simulink model "sf_clutch_enabled_subsystems"  (R2025b)
settings: Solver=ode23  StartTime=0.0  StopTime=10  RelTol=1e-6  AbsTol=1e-7
model workspace (MATLAB code in the model file + MAT data in the model file):
  Fn = [0  0; 1  0.8; 2  1.6; 3  1.6; 4  1.6; 5  1.6; 6  0.8; 7  0; 8  0; 9  0; 10  0]
  Ie = 1
  Iv = 5
  R = 1
  Tin = [1  2; 2  2; 3  2; 4  2; 5  2; 6  0; 7  0; 8  0; 9  0; 10  0]
  be = 2
  bv = 1
  f1 = [1; 6; 11; 16; 21; 26; 31; 36; 41; 46; 51]
  muk = 1
  mus = 1.5
  other statements: load sldemo_clutchparam;
settings Model: ExtModeTrigMode=oneshot  ExtModeArmWhenConnect=off  ExtModeAutoUpdateStatusClock=off  Creator=The MathWorks, Inc.  LastModifiedBy=The MathWorks, Inc.
settings SolverCC: AutoScaleAbsTol=off  AlgebraicLoopSolver=TrustRegion  InsertRTBMode=Auto
settings DataIOCC: ExternalInput=[]  InitialState=[]  SaveFormat=Array  SaveOutput=off  SaveTime=off  ReturnWorkspaceOutputs=off  StateSaveName=x  TimeSaveName=t  OutputSaveName=y  SignalLoggingName=sldemo_clutch_output
settings OptimizationCC: BlockReduction=off  BooleanDataType=off  ReuseModelBlockBuffer=off  ExpressionDepthLimit=2147483647.0  InitFltsAndDblsToZero=on  EfficientMapNaN2IntZero=off  LifeSpan=inf  BufferReusableBoundary=off
settings DebuggingCC: SaveWithParameterizedLinksMsg=none  UnderspecifiedInitializationDetection=Classic  MergeDetectMultiDrivingBlocksExec=none  SignalResolutionControl=TryResolveAllWithWarning  MultiTaskDSMMsg=warning  MultiTaskCondExecSysMsg=none  SigSpecEnsureSampleTimeMsg=none  IntegerOverflowMsg=none  FcnCallInpInsideContextMsg=warning  UnconnectedInputMsg=warning  UnconnectedOutputMsg=warning  UnconnectedLineMsg=warning  BusObjectLabelMismatch=none  StateNameClashWarn=warning  SFUnexpectedBacktrackingDiag=warning  SFNoUnconditionalDefaultTransitionDiag=warning  SFExecutionAtInitializationDiag=none  IntegerSaturationMsg=none  ArithmeticOperatorsInVariantConditions=warning
settings HardwareCC: ProdBitPerPointer=32.0  ProdBitPerSizeT=32.0  ProdBitPerPtrDiffT=32.0  ProdLargestAtomicFloat=None  ProdIntDivRoundTo=Undefined  ProdEndianess=Unspecified  ProdWordSize=32.0  ProdHWDeviceType=32-bit Generic  TargetUnknown=on
settings ModelReferenceCC: EnableRefExpFcnMdlSchedulingChecks=on  PropagateSignalLabelsOutOfModel=off
settings SFSimCC: SFSimEcho=off  SimUseLocalCustomCode=off  SimParseCustomCode=off  CustomCodeUndefinedFunction=UseInterfaceOnly
settings RTWCC: RTWUseLocalCustomCode=off  GPUComputeCapability=3.5
settings CodeAppCC: StateflowObjectComments=on
settings GRTTargetCC: TargetFcnLib=ansi_tfl_tmw.mat  TargetLangStandard=C89/C90 (ANSI)  CombineOutputUpdateFcns=off  GRTInterface=on
settings ConfigComp: CovMetricSettings=d  CovSaveCumulativeToWorkspaceVar=on  CovSaveSingleToWorkspaceVar=on  CovExternalEMLEnable=off

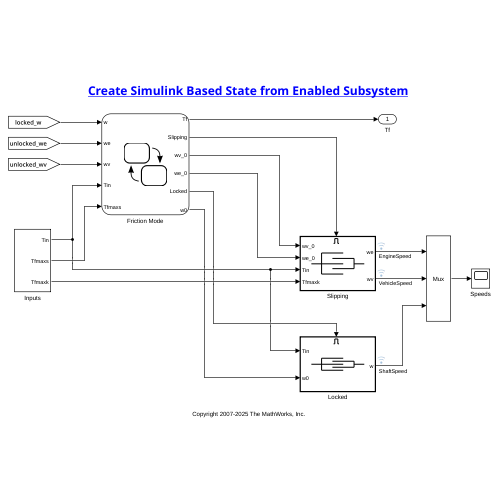
[thumbnail: Simulink's stored preview of the top-level diagram]
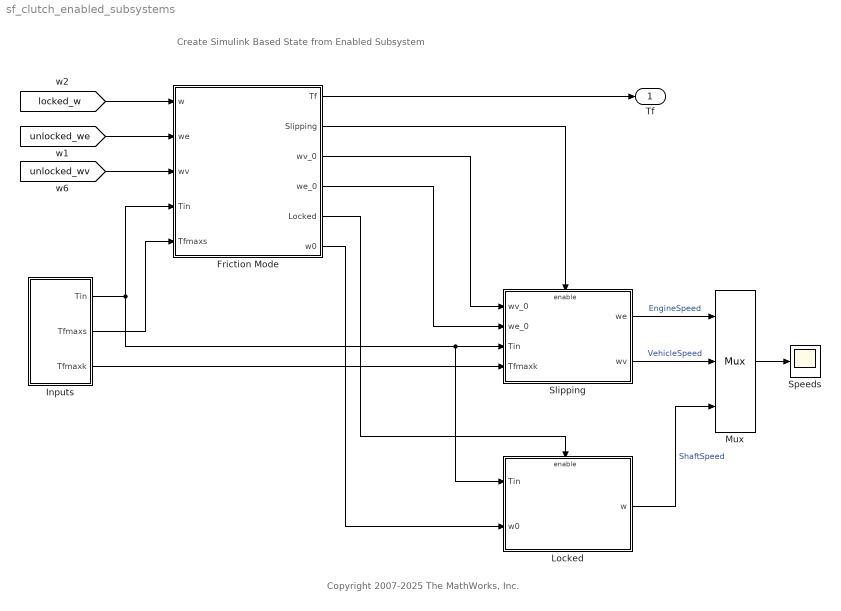
== system sf_clutch_enabled_subsystems ==
  note: Copyright 2007-2025 The MathWorks, Inc.
  note: Create Simulink Based State from Enabled Subsystem
  Friction Mode : Stateflow chart  TreatAsAtomicUnit=on
  Inputs : Subsystem
  Locked : Subsystem  TreatAsAtomicUnit=on
      mask Display: plot(-1,-6,6,12,[0 3],[3 3],[3 1 1 3], [1 1 5 5],[2 4 4 2],[4 4 2 2],[4 5],[3 3])
  Mux : Mux  Inputs=3
  Slipping : Subsystem  TreatAsAtomicUnit=on
      mask Display: plot(-1,-2,6,8,[0 3],[3 3],[3 1 1 3], [1 1 5 5],[2 4 4 2],[4 4 2 2],[4 5],[3 3])
  Speeds : Scope
      settings: TimeSpan=10
  Tf : Outport  InitialOutput=0  VectorParamsAs1DForOutWhenUnconnected=off
  wires:
  [locked_w] -> Friction Mode/1(w)
  [unlocked_we] -> Friction Mode/2(we)
  [unlocked_wv] -> Friction Mode/3(wv)
  Friction Mode/1(Tf) -> Tf/1
  Friction Mode/2(" Slipping") -> Slipping/Enable
  Friction Mode/5(" Locked") -> Locked/Enable
  Friction Mode/6(w0) -> Locked/2(w0)
  Friction Mode/3(wv_0) -> Slipping/1(wv_0)
  Friction Mode/4(we_0) -> Slipping/2(we_0)
  Inputs/1(Tin) -> Friction Mode/4(Tin), Slipping/3(Tin), Locked/1(Tin)
  Inputs/2(Tfmaxs) -> Friction Mode/5(Tfmaxs)
  Inputs/3(Tfmaxk) -> Slipping/4(Tfmaxk)
  Slipping/1(we) -> Mux/1  "EngineSpeed"
  Slipping/2(wv) -> Mux/2  "VehicleSpeed"
  Locked/1(w) -> Mux/3  "ShaftSpeed"
  Mux/1 -> Speeds/1

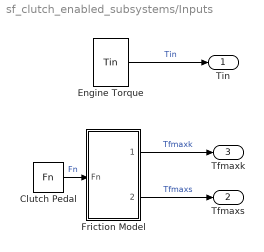
== system sf_clutch_enabled_subsystems/Inputs ==
  Clutch Pedal : FromWorkspace  VariableName=Fn  ZeroCross=off
  Engine Torque : FromWorkspace  VariableName=Tin  ZeroCross=off
  Friction Model : Subsystem
  Tin : Outport  VectorParamsAs1DForOutWhenUnconnected=off
  Tfmaxs : Outport  Port=2  VectorParamsAs1DForOutWhenUnconnected=off
  Tfmaxk : Outport  Port=3  VectorParamsAs1DForOutWhenUnconnected=off
  wires:
  Clutch Pedal/1 -> Friction Model/1(Fn)  "Fn"
  Engine Torque/1 -> Tin/1  "Tin"
  Friction Model/1(Tfmaxk) -> Tfmaxk/1  "Tfmaxk"
  Friction Model/2(Tfmaxs) -> Tfmaxs/1  "Tfmaxs"

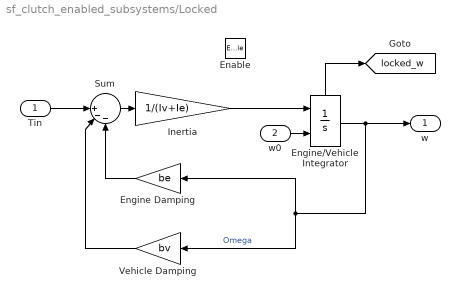
== system sf_clutch_enabled_subsystems/Locked ==
  Tin : Inport
  w0 : Inport  Port=2
  Enable : EnablePort  StatesWhenEnabling=reset
  Engine Damping : Gain  Gain=be  SaturateOnIntegerOverflow=on  OutDataTypeStr=Inherit: Same as input  ParamDataTypeStr=Inherit: Same as input
  Engine/Vehicle Integrator : Integrator  InitialConditionSource=external  ShowStatePort=on
  Inertia : Gain  Gain=1/(Iv+Ie)  SaturateOnIntegerOverflow=on  OutDataTypeStr=Inherit: Same as input  ParamDataTypeStr=Inherit: Same as input
  Sum : Sum  Inputs=||+--  InputSameDT=on  SaturateOnIntegerOverflow=on  OutDataTypeStr=Inherit: Same as first input
  Vehicle Damping : Gain  Gain=bv  SaturateOnIntegerOverflow=on  OutDataTypeStr=Inherit: Same as input  ParamDataTypeStr=Inherit: Same as input
  w : Outport  InitialOutput=0  VectorParamsAs1DForOutWhenUnconnected=off
  tag scope: locked_w=global
  wires:
  w0/1 -> Engine/Vehicle Integrator/2
  Engine/Vehicle Integrator/State -> [locked_w]
  Sum/1 -> Inertia/1
  Tin/1 -> Sum/1
  Engine/Vehicle Integrator/1 -> w/1, Engine Damping/1, Vehicle Damping/1  "Omega"
  Engine Damping/1 -> Sum/3
  Inertia/1 -> Engine/Vehicle Integrator/1
  Vehicle Damping/1 -> Sum/2

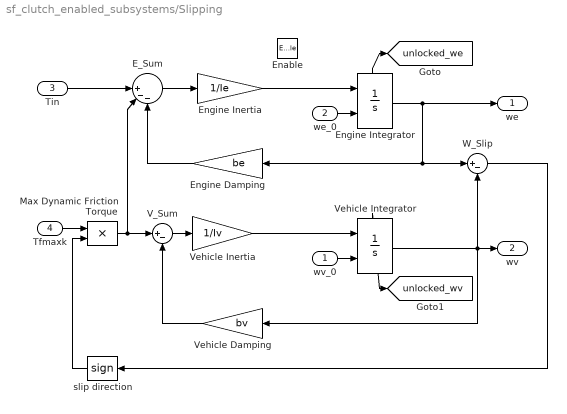
== system sf_clutch_enabled_subsystems/Slipping ==
  wv_0 : Inport
  we_0 : Inport  Port=2
  Tin : Inport  Port=3
  Tfmaxk : Inport  Port=4
  Enable : EnablePort  StatesWhenEnabling=reset
  E_Sum : Sum  Inputs=||+--  InputSameDT=on  SaturateOnIntegerOverflow=on  OutDataTypeStr=Inherit: Same as first input
  Engine Damping : Gain  Gain=be  SaturateOnIntegerOverflow=on  OutDataTypeStr=Inherit: Same as input  ParamDataTypeStr=Inherit: Same as input
  Engine Inertia : Gain  Gain=1/Ie  SaturateOnIntegerOverflow=on  OutDataTypeStr=Inherit: Same as input  ParamDataTypeStr=Inherit: Same as input
  Engine Integrator : Integrator  InitialConditionSource=external  ShowStatePort=on
  Max Dynamic Friction Torque : Product  InputSameDT=on  RndMeth=Zero  SaturateOnIntegerOverflow=on  OutDataTypeStr=Inherit: Same as first input
  V_Sum : Sum  Inputs=|+-  InputSameDT=on  SaturateOnIntegerOverflow=on  OutDataTypeStr=Inherit: Same as first input
  Vehicle Damping : Gain  Gain=bv  SaturateOnIntegerOverflow=on  OutDataTypeStr=Inherit: Same as input  ParamDataTypeStr=Inherit: Same as input
  Vehicle Inertia : Gain  Gain=1/Iv  SaturateOnIntegerOverflow=on  OutDataTypeStr=Inherit: Same as input  ParamDataTypeStr=Inherit: Same as input
  Vehicle Integrator : Integrator  InitialConditionSource=external  ShowStatePort=on
  W_Slip : Sum  Inputs=|+-  InputSameDT=on  SaturateOnIntegerOverflow=on  OutDataTypeStr=Inherit: Same as first input
  slip direction : Signum
  we : Outport  InitialOutput=0  VectorParamsAs1DForOutWhenUnconnected=off
  wv : Outport  Port=2  InitialOutput=0  VectorParamsAs1DForOutWhenUnconnected=off
  tag scope: unlocked_we=global, unlocked_wv=global
  wires:
  V_Sum/1 -> Vehicle Inertia/1
  Vehicle Damping/1 -> V_Sum/2
  Max Dynamic Friction Torque/1 -> V_Sum/1, E_Sum/2
  Tfmaxk/1 -> Max Dynamic Friction Torque/1
  slip direction/1 -> Max Dynamic Friction Torque/2
  W_Slip/1 -> slip direction/1
  Engine Integrator/State -> [unlocked_we]
  Engine Inertia/1 -> Engine Integrator/1
  E_Sum/1 -> Engine Inertia/1
  Engine Damping/1 -> E_Sum/3
  Engine Integrator/1 -> we/1, Engine Damping/1, W_Slip/1
  we_0/1 -> Engine Integrator/2
  Tin/1 -> E_Sum/1
  Vehicle Integrator/State -> [unlocked_wv]
  wv_0/1 -> Vehicle Integrator/2
  Vehicle Inertia/1 -> Vehicle Integrator/1
  Vehicle Integrator/1 -> Vehicle Damping/1, wv/1, W_Slip/2

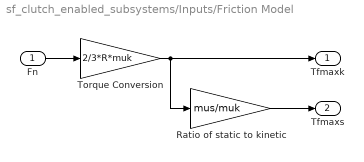
== system sf_clutch_enabled_subsystems/Inputs/Friction Model ==
  Fn : Inport
  Ratio of static to kinetic : Gain  Gain=mus/muk  SaturateOnIntegerOverflow=on  OutDataTypeStr=Inherit: Same as input  ParamDataTypeStr=Inherit: Same as input
  Torque Conversion : Gain  Gain=2/3*R*muk  SaturateOnIntegerOverflow=on  OutDataTypeStr=Inherit: Same as input  ParamDataTypeStr=Inherit: Same as input
  Tfmaxk : Outport  InitialOutput=0  VectorParamsAs1DForOutWhenUnconnected=off
  Tfmaxs : Outport  Port=2  InitialOutput=0  VectorParamsAs1DForOutWhenUnconnected=off
  wires:
  Torque Conversion/1 -> Tfmaxk/1, Ratio of static to kinetic/1
  Fn/1 -> Torque Conversion/1
  Ratio of static to kinetic/1 -> Tfmaxs/1

== stateflow chart sf_clutch_enabled_subsystems/Friction Mode ==
  settings: updateMethod=CONTINUOUS
  state Slipping
    du:
    Tf = getSlipTorque();
    state lockup = detectLockup [function]
      (default) -> (junction 35) : {lockup = (abs(getSlipTorque()) < Tfmaxs) && ...
          |                   in(SlipCalc.SameVelocity);}
    state SlipCalc
      state EngineSlower
      state EngineFaster
      state SameVelocity
      (default) -> (junction 33)
      (junction 33) -> (junction 34) [order 2]
      (junction 34) -> (junction 30) [order 2]
      (junction 34) -> SameVelocity [order 1] : [we == wv]
      (junction 33) -> EngineFaster [order 1] : [we > wv]
      (junction 30) -> EngineSlower
      SameVelocity -> EngineFaster [order 2] : [we > wv]
      SameVelocity -> EngineSlower [order 1] : [we < wv]
      EngineSlower -> SameVelocity : [we >= wv]
      EngineFaster -> SameVelocity : [we <= wv]
  state T = getSlipTorque [function]
    (default) -> (junction 29) : {T = (Tin - we*(be+bv))*Iv/(Iv+Ie)+bv*we;}
  state T = getLockedTorque [function]
    (default) -> (junction 31) : {T = (Iv*Tin-(Iv*be-Ie*bv)*w)/(Iv+Ie);}
  state break = detectSlip [function]
    (default) -> (junction 32) : {break = abs(getLockedTorque()) > Tfmaxs; }
  state Locked
    du:
    Tf = getLockedTorque();
  (default) -> Slipping
  Slipping -> Locked : [Slipping.detectLockup()]
      | {w0 = we;}
  Locked -> Slipping : [detectSlip()]
      | {we_0 = w; wv_0 = w;}
  data: lockup function_output double; T function_output double; T function_output double; break function_output double; Tf output double; Slipping output boolean; wv_0 output double; we_0 output double; Locked output boolean; w input double; we input double; wv input double; Tin input double; Tfmaxs input double; be parameter double; bv parameter double; Ie parameter double; Iv parameter double; w0 output double
